simulink model "ExpS6_TwoR_armPIDControl_CTCTraj"  (R2022b)
settings: Solver=VariableStepAuto  StartTime=0.0  StopTime=10.0  RelTol=1e-3
undefined symbols (not defined in the file): X, Y, Z
libraries: sm_lib x16, nesl_utility x11, robotmaniplib x4, simulink_extras x4, robotcorelib x1
settings Model: Creator=HP  LastModifiedBy=amrita

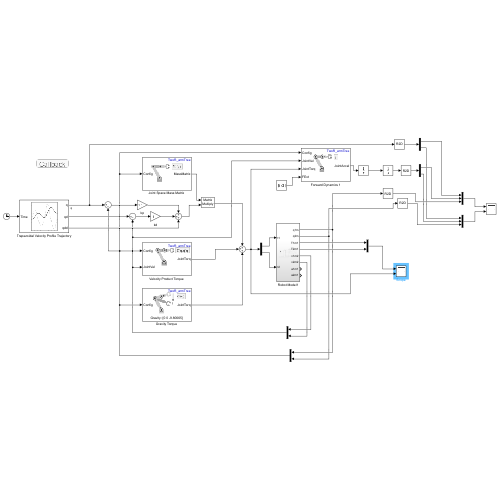
[thumbnail: Simulink's stored preview of the top-level diagram]
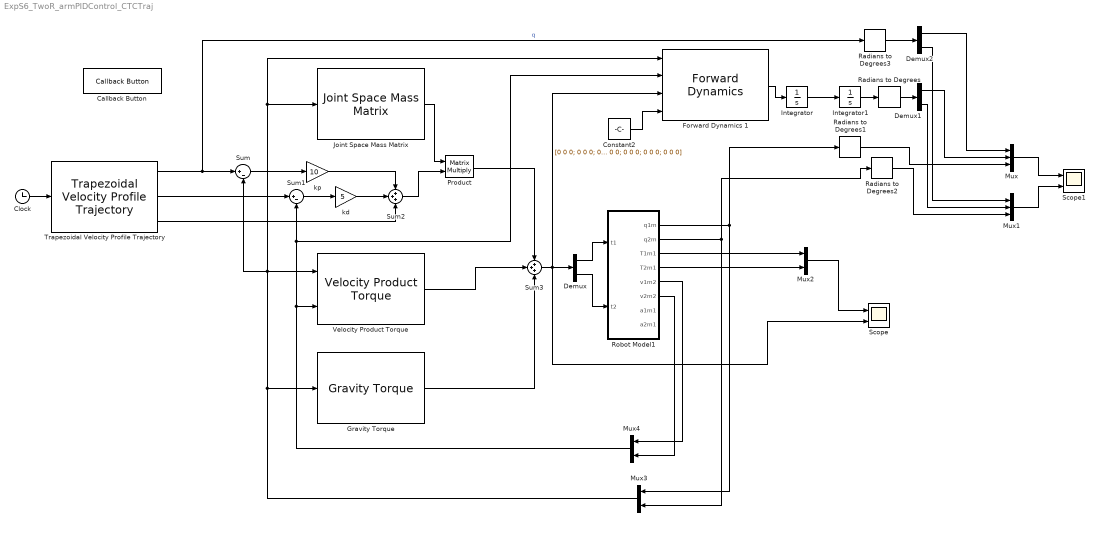
== system ExpS6_TwoR_armPIDControl_CTCTraj ==
  Callback Button : CallbackButton
      settings: ClickFcn=|
      | [TwoR_armTree, TwoR_armInfo] = importrobot('ExpS1a_TwoR_armModel.slx');
      | %t = [0 1 4 ];
      | q1 = [0 0 0 90 90]*pi/180;
      | q2 = [0 0 0 -360 -360]*pi/180;%[360 360 360 0 0]*pi/180;
      | v1 = [ 0 15 15 0; 0 60 60 0]; %
      | %Waypoints set 1
      | wp1 = [q1;q2];
  Clock : Clock
  Constant2 : Constant  Value=[0 0 0; 0 0 0; 0 0 0; 0 0 0; 0 0 0; 0 0 0]
  Demux : Demux  Outputs=2
  Demux1 : Demux  Outputs=2
  Demux2 : Demux  Outputs=2
  Forward Dynamics 1 : robotmaniplib/Forward Dynamics  RigidBodyTree=TwoR_armTree  SimulateUsing=Interpreted execution
  "Gravity Torque " : robotmaniplib/Gravity Torque  RigidBodyTree=TwoR_armTree  SimulateUsing=Interpreted execution
  Integrator : Integrator
  Integrator1 : Integrator
  "Joint Space Mass Matrix " : robotmaniplib/Joint Space Mass Matrix  RigidBodyTree=TwoR_armTree  SimulateUsing=Interpreted execution
  Mux : Mux  Inputs=3
  Mux1 : Mux  Inputs=3
  Mux2 : Mux  Inputs=2
  Mux3 : Mux  Inputs=2
  Mux4 : Mux  Inputs=2
  Product : Product  Multiplication=Matrix(*)
  Radians to Degrees{,1..3} (4 alike) : simulink_extras/Transformations/Radians to Degrees
  Robot Model1 : Subsystem
  Scope : Scope  NumInputPorts=2
  Scope1 : Scope  NumInputPorts=2
  Sum : Sum  Inputs=|+-
  Sum1 : Sum  Inputs=|+-
  Sum2 : Sum  Inputs=+++
  Sum3 : Sum  Inputs=+++
  Trapezoidal Velocity Profile Trajectory : robotcorelib/Trapezoidal Velocity Profile Trajectory  WaypointSource=Internal  Waypoints=wp1  NumParams=1  Parameter1=Peak Velocity  Parameter2=Acceleration Time  ParameterSource=Internal  PeakVelocity=vp1  Acceleration=acc  EndTime=[ 1; 1 ]  AccelTime=acct  SimulateUsing=Interpreted execution
  "Velocity Product Torque " : robotmaniplib/Velocity Product Torque  RigidBodyTree=TwoR_armTree  SimulateUsing=Interpreted execution
  kd : Gain  Gain=5
  kp : Gain  Gain=10
  wires:
  Clock/1 -> Trapezoidal Velocity Profile Trajectory/1
  Forward Dynamics 1/1 -> Integrator/1
  Integrator/1 -> Integrator1/1
  Robot Model1/4(T2m1) -> Mux2/2
  Robot Model1/3(T1m1) -> Mux2/1
  Integrator1/1 -> Radians to Degrees/1
  Radians to Degrees/1 -> Demux1/1
  Demux2/1 -> Mux/1
  Demux1/1 -> Mux/2
  Radians to Degrees1/1 -> Mux/3
  Radians to Degrees2/1 -> Mux1/3
  Demux1/2 -> Mux1/2
  Demux2/2 -> Mux1/1
  Mux/1 -> Scope1/1
  Mux1/1 -> Scope1/2
  Robot Model1/1(q1m) -> Radians to Degrees1/1, Mux3/1
  Robot Model1/2(q2m) -> Radians to Degrees2/1, Mux3/2
  Robot Model1/6(v2m2) -> Mux4/2
  Robot Model1/5(v1m2) -> Mux4/1
  Trapezoidal Velocity Profile Trajectory/1 -> Radians to Degrees3/1, Sum/1  "q"
  Mux3/1 -> Forward Dynamics 1/1, "Joint Space Mass Matrix "/1, Sum/2, "Velocity Product Torque "/1, "Gravity Torque "/1
  Trapezoidal Velocity Profile Trajectory/2 -> Sum1/1
  Mux4/1 -> "Velocity Product Torque "/2, Forward Dynamics 1/2, Sum1/2
  Sum/1 -> kp/1
  Sum1/1 -> kd/1
  kp/1 -> Sum2/1
  kd/1 -> Sum2/2
  Trapezoidal Velocity Profile Trajectory/3 -> Sum2/3
  "Joint Space Mass Matrix "/1 -> Product/1
  Sum2/1 -> Product/2
  Product/1 -> Sum3/1
  "Velocity Product Torque "/1 -> Sum3/2
  "Gravity Torque "/1 -> Sum3/3
  Demux/1 -> Robot Model1/1(t1)
  Demux/2 -> Robot Model1/2(t2)
  Mux2/1 -> Scope/1
  Sum3/1 -> Forward Dynamics 1/3, Scope/2, Demux/1
  Constant2/1 -> Forward Dynamics 1/4
  Radians to Degrees3/1 -> Demux2/1

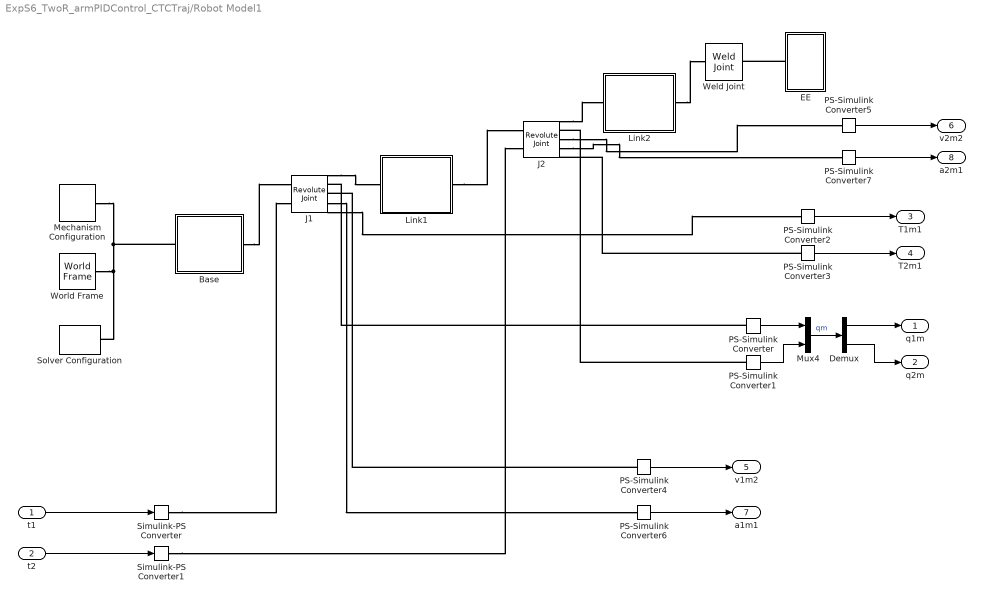
== system ExpS6_TwoR_armPIDControl_CTCTraj/Robot Model1 ==
  t1 : Inport
  t2 : Inport  Port=2
  Base : Subsystem
  Demux : Demux  Outputs=2
  EE : Subsystem
  J1 : sm_lib/Joints/Revolute Joint  JointMode=Normal  SenseConstraintForce=off  SenseConstraintForceX=off  SenseConstraintForceY=off  SenseConstraintForceZ=off  SenseConstraintTorque=off  SenseConstraintTorqueX=off  SenseConstraintTorqueY=off  SenseConstraintTorqueZ=off  SenseTotalForce=off  SenseTotalForceX=off  SenseTotalForceY=off  SenseTotalForceZ=off  SenseTotalTorque=off  SenseTotalTorqueX=off  SenseTotalTorqueY=off  SenseTotalTorqueZ=off  CompositeWrenchDir=FollowerOnBase  CompositeWrenchFrame=BaseFrame  EquilibriumPosition=0  EquilibriumPositionUnits=deg  SpringStiffness=0  SpringStiffnessUnits=N*m/deg  DampingCoefficient=0  DampingCoefficientUnits=N*m/(deg/s)  TorqueActuationMode=InputTorque  MotionActuationMode=ComputedMotion  SensePosition=on  SenseVelocity=on  SenseAcceleration=on  SenseTorqueForce=on  SenseLowerLimitTorqueForce=off  SenseUpperLimitTorqueForce=off  LowerLimitSpecify=off  LowerLimitBound=-270  LowerLimitBoundUnits=deg  LowerLimitStiffness=1e4  LowerLimitStiffnessUnits=N*m/deg  LowerLimitDamping=10  LowerLimitDampingUnits=N*m/(deg/s)  LowerLimitTransitionRegionWidth=0.1  LowerLimitTransitionRegionWidthUnits=deg  UpperLimitSpecify=off  UpperLimitBound=-180  UpperLimitBoundUnits=deg  UpperLimitStiffness=1e4  UpperLimitStiffnessUnits=N*m/deg  UpperLimitDamping=10  UpperLimitDampingUnits=N*m/(deg/s)  UpperLimitTransitionRegionWidth=0.1  UpperLimitTransitionRegionWidthUnits=deg  PositionTargetSpecify=off  PositionTargetPriority=High  PositionTargetValue=0  PositionTargetValueUnits=deg  VelocityTargetSpecify=off  VelocityTargetPriority=High  VelocityTargetValue=0  VelocityTargetValueUnits=deg/s
  J2 : sm_lib/Joints/Revolute Joint  JointMode=Normal  SenseConstraintForce=off  SenseConstraintForceX=off  SenseConstraintForceY=off  SenseConstraintForceZ=off  SenseConstraintTorque=off  SenseConstraintTorqueX=off  SenseConstraintTorqueY=off  SenseConstraintTorqueZ=off  SenseTotalForce=off  SenseTotalForceX=off  SenseTotalForceY=off  SenseTotalForceZ=off  SenseTotalTorque=off  SenseTotalTorqueX=off  SenseTotalTorqueY=off  SenseTotalTorqueZ=off  CompositeWrenchDir=FollowerOnBase  CompositeWrenchFrame=BaseFrame  EquilibriumPosition=0  EquilibriumPositionUnits=deg  SpringStiffness=0  SpringStiffnessUnits=N*m/deg  DampingCoefficient=0  DampingCoefficientUnits=N*m/(deg/s)  TorqueActuationMode=InputTorque  MotionActuationMode=ComputedMotion  SensePosition=on  SenseVelocity=on  SenseAcceleration=on  SenseTorqueForce=on  SenseLowerLimitTorqueForce=off  SenseUpperLimitTorqueForce=off  LowerLimitSpecify=off  LowerLimitBound=0  LowerLimitBoundUnits=deg  LowerLimitStiffness=1e4  LowerLimitStiffnessUnits=N*m/deg  LowerLimitDamping=10  LowerLimitDampingUnits=N*m/(deg/s)  LowerLimitTransitionRegionWidth=0.1  LowerLimitTransitionRegionWidthUnits=deg  UpperLimitSpecify=off  UpperLimitBound=360  UpperLimitBoundUnits=deg  UpperLimitStiffness=1e4  UpperLimitStiffnessUnits=N*m/deg  UpperLimitDamping=10  UpperLimitDampingUnits=N*m/(deg/s)  UpperLimitTransitionRegionWidth=0.1  UpperLimitTransitionRegionWidthUnits=deg  PositionTargetSpecify=off  PositionTargetPriority=High  PositionTargetValue=0  PositionTargetValueUnits=deg  VelocityTargetSpecify=off  VelocityTargetPriority=High  VelocityTargetValue=0  VelocityTargetValueUnits=deg/s
  Link1 : Subsystem
  Link2 : Subsystem
  Mechanism Configuration : sm_lib/Utilities/Mechanism Configuration  UniformGravity=Constant  GravityVector=[0 0 -9.80665]  GravityUnits=m/s^2  LinearizationDelta=0.001  JointModeTransitionNonlinearIterations=2
  Mux4 : Mux  Inputs=2
  PS-Simulink Converter{,1..7} (8 alike) : nesl_utility/PS-Simulink Converter  PhysicalDomain=network_engine_domain  SubClassName=ps_output  LeftPortType=input  RightPortType=output  PseudoPeriodic=off  Frequencies=[]  VectorFormat=inherit  Unit=inherit  AffineConversion=off
  Simulink-PS Converter : nesl_utility/Simulink-PS Converter  PhysicalDomain=network_engine_domain  SubClassName=ps_input  LeftPortType=input  RightPortType=output  PseudoPeriodic=off  Frequencies=[]  NoiseDistribution=none  NoiseParameters=[]  Unit=N*m  AffineConversion=off  FilteringAndDerivatives=provide  SimscapeFilterOrder=1  InputFilterTimeConstant=0.001  UdotUserProvided=0
  Simulink-PS Converter1 : nesl_utility/Simulink-PS Converter  PhysicalDomain=network_engine_domain  SubClassName=ps_input  LeftPortType=input  RightPortType=output  PseudoPeriodic=off  Frequencies=[]  NoiseDistribution=none  NoiseParameters=[]  Unit=N*m  AffineConversion=off  FilteringAndDerivatives=provide  SimscapeFilterOrder=1  InputFilterTimeConstant=0.001  UdotUserProvided=0
  Solver Configuration : nesl_utility/Solver Configuration  PhysicalDomain=network_engine_domain  SubClassName=solver  LeftPortType=input  RightPortType=generic  Tones=[]  Harmonics=[]  SimulateNoise=off  Profile=off  UseLocalSampling=off  EnableSwitchedLinearOptims=on  FrequencyDomain=off  UseCCode=off  RelTol=0.001  AbsTol=0.001  MinStep=1e-09  ToWorkspace=off  RevertToSquareIcSolve=off  NumHomotopyIterations=100  PhasorMode=off  PhasorModeNumHarmonics=1  ConsistencySolver=NEWTON_XTOL_AFTER_FTOL  IndexReductionMethod=DerivativeReplacement  DoDC=off  ResidualTolerance=1e-09  ConsistencyTolSource=GLOBAL  ConsistencyAbsTol=0.001  ConsistencyRelTol=0.001  ConsistencyTolFactor=0.001  UseLocalSolver=off  LocalSolverChoice=NE_BACKWARD_EULER_ADVANCER  ResolveIndetEquations=on  FunctionEvalNumThread=1  LocalSolverSampleTime=0.001  DoFixedCost=off  MaxNonlinIter=3  MaxModeIter=2  ComputeImpulses=off  ImpulseIterations=2  LinearAlgebra=auto  LinearAlgebraNumThread=0  EquationFormulation=NE_TIME_EF  DelaysMemoryBudget=1024  AutomaticFiltering=on  FilteringTimeConstant=0.001  PartitionStorageMethod=AS_NEEDED  PartitionMemoryBudget=1024  PartitionMethod=ROBUST
  Weld Joint : sm_lib/Joints/Weld Joint  JointMode=Normal  SenseConstraintForce=off  SenseConstraintForceX=off  SenseConstraintForceY=off  SenseConstraintForceZ=off  SenseConstraintTorque=off  SenseConstraintTorqueX=off  SenseConstraintTorqueY=off  SenseConstraintTorqueZ=off  SenseTotalForce=off  SenseTotalForceX=off  SenseTotalForceY=off  SenseTotalForceZ=off  SenseTotalTorque=off  SenseTotalTorqueX=off  SenseTotalTorqueY=off  SenseTotalTorqueZ=off  CompositeWrenchDir=FollowerOnBase  CompositeWrenchFrame=BaseFrame
  World Frame : sm_lib/Frames and Transforms/World Frame
  q1m : Outport
  q2m : Outport  Port=2
  T1m1 : Outport  Port=3
  T2m1 : Outport  Port=4
  v1m2 : Outport  Port=5
  v2m2 : Outport  Port=6
  a1m1 : Outport  Port=7
  a2m1 : Outport  Port=8
  wires:
  PS-Simulink Converter6/1 -> a1m1/1
  PS-Simulink Converter7/1 -> a2m1/1
  PS-Simulink Converter5/1 -> v2m2/1
  PS-Simulink Converter4/1 -> v1m2/1
  PS-Simulink Converter2/1 -> T1m1/1
  PS-Simulink Converter3/1 -> T2m1/1
  t2/1 -> Simulink-PS Converter1/1
  t1/1 -> Simulink-PS Converter/1
  Mux4/1 -> Demux/1  "qm"
  Demux/1 -> q1m/1
  Demux/2 -> q2m/1
  PS-Simulink Converter/1 -> Mux4/1
  PS-Simulink Converter1/1 -> Mux4/2
  connections:
  J2/RConn4 -- PS-Simulink Converter7/LConn1
  J2/RConn3 -- PS-Simulink Converter5/LConn1
  J1/RConn4 -- PS-Simulink Converter6/LConn1
  PS-Simulink Converter4/LConn1 -- J1/RConn3
  PS-Simulink Converter3/LConn1 -- J2/RConn5
  J1/RConn5 -- PS-Simulink Converter2/LConn1
  Link1/RConn1 -- J2/LConn1
  J1/RConn1 -- Link1/LConn1
  Link2/RConn1 -- Weld Joint/LConn1
  J2/RConn1 -- Link2/LConn1
  EE/LConn1 -- Weld Joint/RConn1
  PS-Simulink Converter1/LConn1 -- J2/RConn2
  Base/RConn1 -- J1/LConn1
  Simulink-PS Converter/RConn1 -- J1/LConn2
  PS-Simulink Converter/LConn1 -- J1/RConn2
  Simulink-PS Converter1/RConn1 -- J2/LConn2
  Base/LConn1 -- Solver Configuration/RConn1 -- World Frame/RConn1 -- Mechanism Configuration/RConn1

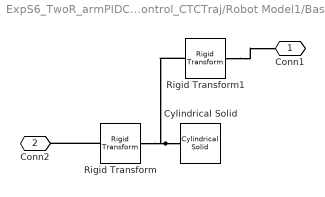
== system ExpS6_TwoR_armPIDControl_CTCTraj/Robot Model1/Base ==
  Cylindrical Solid : sm_lib/Body Elements/Cylindrical Solid  GraphicAmbientColor=[0.15 0.15 0.15 1.0]  BasedOnType=Density  CenterOfMass=[0 0 0]  CenterOfMassUnits=m  GraphicDiffuseColor=[0.0 0.0 1.0]  CylinderLength=0.2  CylinderLengthUnits=m  CylinderRadius=0.05  CylinderRadiusUnits=m  Density=1000  DensityUnits=kg/m^3  DoExposeReferenceFrame=on  GraphicEmissiveColor=[0.0 0.0 0.0 1.0]  ExportEntireGeometry=off  SerializedFrames=<Frames/>  MarkerShape=Sphere  MarkerSize=10  GraphicType=FromGeometry  InertiaType=CalculateFromGeometry  Mass=1  MassUnits=kg  MomentsOfInertia=[1 1 1]  MomentsOfInertiaUnits=kg*m^2  GraphicOpacity=1.0  ProductsOfInertia=[0 0 0]  ProductsOfInertiaUnits=kg*m^2  GraphicShininess=75  GraphicSpecularColor=[0.5 0.5 0.5 1.0]  GraphicVisPropType=SimpleVisualProperties
  Rigid Transform : sm_lib/Frames and Transforms/Rigid Transform  TranslationMethod=Cartesian  TranslationStandardOffset=0  TranslationLengthUnit=m  TranslationStandardAxis=+Z  TranslationCartesianOffset=[0 0 0.1]  TranslationROffset=0  TranslationROffsetUnits=m  TranslationZOffset=0  TranslationZOffsetUnits=m  TranslationThetaOffset=0  TranslationThetaOffsetUnits=deg  RotationMethod=None  RotationAngleUnits=deg  RotationStandardAxis=+Z  RotationAngle=0.0  RotationArbitraryAxis=[0 0 1]  FollAlignAxisA=+X  BaseAlignAxisA=+Y  FollAlignAxisB=+Y  BaseAlignAxisB=+Z  RotationSequenceAxes=FollowerAxes  RotationSequence=XYX  RotationSequenceAngles=[0 0 0]  RotationSequenceAnglesUnits=deg  RotationMatrix=[1 0 0; 0 1 0; 0 0 1]  Quaternion=[1 0 0 0]
  Rigid Transform1 : sm_lib/Frames and Transforms/Rigid Transform  TranslationMethod=Cartesian  TranslationStandardOffset=0  TranslationLengthUnit=m  TranslationStandardAxis=+Z  TranslationCartesianOffset=[0 0 0.1]  TranslationROffset=0  TranslationROffsetUnits=m  TranslationZOffset=0  TranslationZOffsetUnits=m  TranslationThetaOffset=0  TranslationThetaOffsetUnits=deg  RotationMethod=None  RotationAngleUnits=deg  RotationStandardAxis=+Z  RotationAngle=0.0  RotationArbitraryAxis=[0 0 1]  FollAlignAxisA=+X  BaseAlignAxisA=+Y  FollAlignAxisB=+Y  BaseAlignAxisB=+Z  RotationSequenceAxes=FollowerAxes  RotationSequence=XYX  RotationSequenceAngles=[0 0 0]  RotationSequenceAnglesUnits=deg  RotationMatrix=[1 0 0; 0 1 0; 0 0 1]  Quaternion=[1 0 0 0]
  Conn1 : PMIOPort  Side=Right
  Conn2 : PMIOPort  Port=2  Side=Left
  connections:
  Rigid Transform/LConn1 -- Conn2/RConn1
  Rigid Transform1/RConn1 -- Conn1/RConn1
  Cylindrical Solid/RConn1 -- Rigid Transform1/LConn1 -- Rigid Transform/RConn1

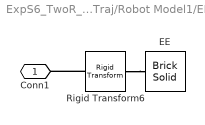
== system ExpS6_TwoR_armPIDControl_CTCTraj/Robot Model1/EE ==
  EE : sm_lib/Body Elements/Brick Solid  GraphicAmbientColor=[0.15 0.15 0.15 1.0]  BasedOnType=Density  BrickDimensions=[0.02 0.02 0.02]  BrickDimensionUnits=m  CenterOfMass=[0 0 0]  CenterOfMassUnits=m  GraphicDiffuseColor=[1.0 0.0 0.0]  Density=1000  DensityUnits=kg/m^3  DoExposeReferenceFrame=on  GraphicEmissiveColor=[0.0 0.0 0.0 1.0]  ExportEntireGeometry=off  SerializedFrames=<Frames/>  MarkerShape=Sphere  MarkerSize=10  GraphicType=FromGeometry  InertiaType=CalculateFromGeometry  Mass=1  MassUnits=kg  MomentsOfInertia=[1 1 1]  MomentsOfInertiaUnits=kg*m^2  GraphicOpacity=1.0  ProductsOfInertia=[0 0 0]  ProductsOfInertiaUnits=kg*m^2  GraphicShininess=75  GraphicSpecularColor=[0.5 0.5 0.5 1.0]  GraphicVisPropType=SimpleVisualProperties
  Rigid Transform6 : sm_lib/Frames and Transforms/Rigid Transform  TranslationMethod=Cartesian  TranslationStandardOffset=0  TranslationLengthUnit=m  TranslationStandardAxis=+Z  TranslationCartesianOffset=[0.01 0 0]  TranslationROffset=0  TranslationROffsetUnits=m  TranslationZOffset=0  TranslationZOffsetUnits=m  TranslationThetaOffset=0  TranslationThetaOffsetUnits=deg  RotationMethod=None  RotationAngleUnits=deg  RotationStandardAxis=+Z  RotationAngle=0.0  RotationArbitraryAxis=[0 0 1]  FollAlignAxisA=+X  BaseAlignAxisA=+Y  FollAlignAxisB=+Y  BaseAlignAxisB=+Z  RotationSequenceAxes=FollowerAxes  RotationSequence=XYX  RotationSequenceAngles=[0 0 0]  RotationSequenceAnglesUnits=deg  RotationMatrix=[1 0 0; 0 1 0; 0 0 1]  Quaternion=[1 0 0 0]
  Conn1 : PMIOPort  Side=Left
  connections:
  Rigid Transform6/LConn1 -- Conn1/RConn1
  Rigid Transform6/RConn1 -- EE/RConn1

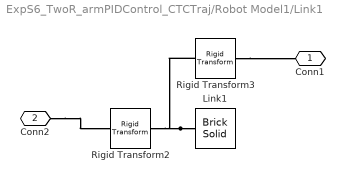
== system ExpS6_TwoR_armPIDControl_CTCTraj/Robot Model1/Link1 ==
  Link1 : sm_lib/Body Elements/Brick Solid  GraphicAmbientColor=[0.15 0.15 0.15 1.0]  BasedOnType=Density  BrickDimensions=[0.6 0.1 0.05]  BrickDimensionUnits=m  CenterOfMass=[0 0 0]  CenterOfMassUnits=m  GraphicDiffuseColor=[1.0 0.4 0.4]  Density=1000  DensityUnits=kg/m^3  DoExposeReferenceFrame=on  GraphicEmissiveColor=[0.0 0.0 0.0 1.0]  ExportEntireGeometry=off  SerializedFrames=<Frames/>  MarkerShape=Sphere  MarkerSize=10  GraphicType=FromGeometry  InertiaType=CalculateFromGeometry  Mass=1  MassUnits=kg  MomentsOfInertia=[1 1 1]  MomentsOfInertiaUnits=kg*m^2  GraphicOpacity=1.0  ProductsOfInertia=[0 0 0]  ProductsOfInertiaUnits=kg*m^2  GraphicShininess=75  GraphicSpecularColor=[0.5 0.5 0.5 1.0]  GraphicVisPropType=SimpleVisualProperties
  Rigid Transform2 : sm_lib/Frames and Transforms/Rigid Transform  TranslationMethod=Cartesian  TranslationStandardOffset=0  TranslationLengthUnit=m  TranslationStandardAxis=+Z  TranslationCartesianOffset=[0.3 0 0.025]  TranslationROffset=0  TranslationROffsetUnits=m  TranslationZOffset=0  TranslationZOffsetUnits=m  TranslationThetaOffset=0  TranslationThetaOffsetUnits=deg  RotationMethod=None  RotationAngleUnits=deg  RotationStandardAxis=+Z  RotationAngle=0.0  RotationArbitraryAxis=[0 0 1]  FollAlignAxisA=+X  BaseAlignAxisA=+Y  FollAlignAxisB=+Y  BaseAlignAxisB=+Z  RotationSequenceAxes=FollowerAxes  RotationSequence=XYX  RotationSequenceAngles=[0 0 0]  RotationSequenceAnglesUnits=deg  RotationMatrix=[1 0 0; 0 1 0; 0 0 1]  Quaternion=[1 0 0 0]
  Rigid Transform3 : sm_lib/Frames and Transforms/Rigid Transform  TranslationMethod=Cartesian  TranslationStandardOffset=0  TranslationLengthUnit=m  TranslationStandardAxis=+Z  TranslationCartesianOffset=[0.3 0 0]  TranslationROffset=0  TranslationROffsetUnits=m  TranslationZOffset=0  TranslationZOffsetUnits=m  TranslationThetaOffset=0  TranslationThetaOffsetUnits=deg  RotationMethod=None  RotationAngleUnits=deg  RotationStandardAxis=+Z  RotationAngle=0.0  RotationArbitraryAxis=[0 0 1]  FollAlignAxisA=+X  BaseAlignAxisA=+Y  FollAlignAxisB=+Y  BaseAlignAxisB=+Z  RotationSequenceAxes=FollowerAxes  RotationSequence=XYX  RotationSequenceAngles=[0 0 0]  RotationSequenceAnglesUnits=deg  RotationMatrix=[1 0 0; 0 1 0; 0 0 1]  Quaternion=[1 0 0 0]
  Conn1 : PMIOPort  Side=Right
  Conn2 : PMIOPort  Port=2  Side=Left
  connections:
  Rigid Transform3/RConn1 -- Conn1/RConn1
  Conn2/RConn1 -- Rigid Transform2/LConn1
  Link1/RConn1 -- Rigid Transform3/LConn1 -- Rigid Transform2/RConn1

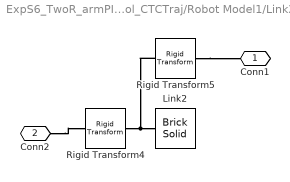
== system ExpS6_TwoR_armPIDControl_CTCTraj/Robot Model1/Link2 ==
  Link2 : sm_lib/Body Elements/Brick Solid  GraphicAmbientColor=[0.15 0.15 0.15 1.0]  BasedOnType=Density  BrickDimensions=[0.4 0.1 0.05]  BrickDimensionUnits=m  CenterOfMass=[0 0 0]  CenterOfMassUnits=m  GraphicDiffuseColor=[0.4 1.0 0.4]  Density=1000  DensityUnits=kg/m^3  DoExposeReferenceFrame=on  GraphicEmissiveColor=[0.0 0.0 0.0 1.0]  ExportEntireGeometry=off  SerializedFrames=<Frames/>  MarkerShape=Sphere  MarkerSize=10  GraphicType=FromGeometry  InertiaType=CalculateFromGeometry  Mass=1  MassUnits=kg  MomentsOfInertia=[1 1 1]  MomentsOfInertiaUnits=kg*m^2  GraphicOpacity=1.0  ProductsOfInertia=[0 0 0]  ProductsOfInertiaUnits=kg*m^2  GraphicShininess=75  GraphicSpecularColor=[0.5 0.5 0.5 1.0]  GraphicVisPropType=SimpleVisualProperties
  Rigid Transform4 : sm_lib/Frames and Transforms/Rigid Transform  TranslationMethod=Cartesian  TranslationStandardOffset=0  TranslationLengthUnit=m  TranslationStandardAxis=+Z  TranslationCartesianOffset=[0.2 0 0.05]  TranslationROffset=0  TranslationROffsetUnits=m  TranslationZOffset=0  TranslationZOffsetUnits=m  TranslationThetaOffset=0  TranslationThetaOffsetUnits=deg  RotationMethod=None  RotationAngleUnits=deg  RotationStandardAxis=+Z  RotationAngle=0.0  RotationArbitraryAxis=[0 0 1]  FollAlignAxisA=+X  BaseAlignAxisA=+Y  FollAlignAxisB=+Y  BaseAlignAxisB=+Z  RotationSequenceAxes=FollowerAxes  RotationSequence=XYX  RotationSequenceAngles=[0 0 0]  RotationSequenceAnglesUnits=deg  RotationMatrix=[1 0 0; 0 1 0; 0 0 1]  Quaternion=[1 0 0 0]
  Rigid Transform5 : sm_lib/Frames and Transforms/Rigid Transform  TranslationMethod=Cartesian  TranslationStandardOffset=0  TranslationLengthUnit=m  TranslationStandardAxis=+Z  TranslationCartesianOffset=[0.2 0 0]  TranslationROffset=0  TranslationROffsetUnits=m  TranslationZOffset=0  TranslationZOffsetUnits=m  TranslationThetaOffset=0  TranslationThetaOffsetUnits=deg  RotationMethod=None  RotationAngleUnits=deg  RotationStandardAxis=+Z  RotationAngle=0.0  RotationArbitraryAxis=[0 0 1]  FollAlignAxisA=+X  BaseAlignAxisA=+Y  FollAlignAxisB=+Y  BaseAlignAxisB=+Z  RotationSequenceAxes=FollowerAxes  RotationSequence=XYX  RotationSequenceAngles=[0 0 0]  RotationSequenceAnglesUnits=deg  RotationMatrix=[1 0 0; 0 1 0; 0 0 1]  Quaternion=[1 0 0 0]
  Conn1 : PMIOPort  Side=Right
  Conn2 : PMIOPort  Port=2  Side=Left
  connections:
  Rigid Transform5/RConn1 -- Conn1/RConn1
  Link2/RConn1 -- Rigid Transform5/LConn1 -- Rigid Transform4/RConn1
  Conn2/RConn1 -- Rigid Transform4/LConn1
